simulink model "aero2_hardware_cascade_R2021a"  (R2021a)
settings: Solver=ode1  StartTime=0.0  StopTime=60  FixedStep=0.002  RelTol=1e-3  EnableMultiTasking=on
model workspace (MAT data in the model file):
  Dq = 2.25
  Kaw = 20
  Kff = 1
  Ki = 1.84164606325
  Kp = 0.216370391856
  Kq = 2.25
  ReferenceRate = [0 0.002 0.004 0.006 0.008 0.01 0.012 0.014 0.016 0.018 0.02 0.022 ... (90003 elements, 30001x3)]
  Ts = 0.002
  U_h : timeseries (value not decoded)
  U_v : timeseries (value not decoded)
  X0 = [0; 0; 0; 0]
  meas_on = 0
undefined symbols (not defined in the file): DiscIntNeverNeededParam, HIL, qc_get_step_size
libraries: quarc_library x4
(part 2 of 2)

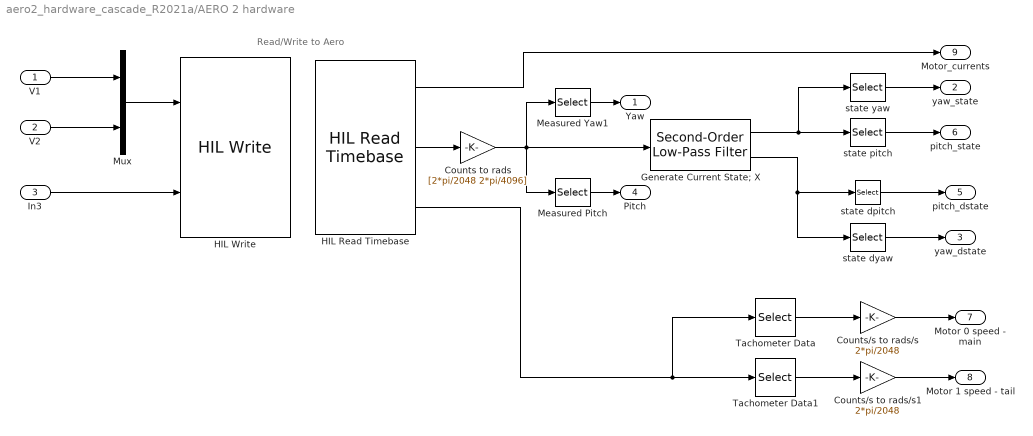
== system aero2_hardware_cascade_R2021a/AERO 2 hardware ==
  note: Read/Write to Aero
  V1 : Inport
  V2 : Inport  Port=2
  In3 : Inport  Port=3
  Counts to rads : Gain  Gain=[2*pi/2048 2*pi/4096]
  Counts/s to rads/s : Gain  Gain=2*pi/2048
  Counts/s to rads/s1 : Gain  Gain=2*pi/2048
  Generate Current State; X : quarc_library/Continuous/Second-Order Low-Pass Filter  params_source=Internal (dialog parameters)  input_width=10  input_zeta=0.8  input_init=0
  HIL Read Timebase : quarc_library/Data Acquisition/Generic/Timebases/HIL Read Timebase  object_name=HIL-1  clock=0  analog_channels=[0:1]  encoder_channels=[2:3]  digital_channels=[]  other_channels=[4000 4002 14000 14001]  active=on  vector_output=on  data_type_mode=Inherit via back propagation  encoder_data_type=double  digital_data_type=boolean  overflow_mode=Error on overflow  samples_in_buffer=max(ceil(1/qc_get_step_size), 1)
  HIL Write : quarc_library/Data Acquisition/Generic/Immediate I//O/HIL Write  object_name=HIL-1  analog_channels=[0:1]  pwm_channels=[]  digital_channels=[]  other_channels=[11000:11002]  sample_time=-1  active=off  vector_input=on
  Measured Pitch : Selector  InputPortWidth=2  IndexOptions=Index vector (dialog)  Indices=[1]  OutputSizes=1
  Measured Yaw1 : Selector  InputPortWidth=2  IndexOptions=Index vector (dialog)  Indices=[2]  OutputSizes=1
  Mux : Mux  Inputs=2
  Tachometer Data : Selector  InputPortWidth=4  IndexOptions=Index vector (dialog)  Indices=[3]  OutputSizes=1
  Tachometer Data1 : Selector  InputPortWidth=4  IndexOptions=Index vector (dialog)  Indices=[4]  OutputSizes=1
  state dpitch : Selector  InputPortWidth=2  IndexOptions=Index vector (dialog)  Indices=[1]  OutputSizes=1
  state dyaw : Selector  InputPortWidth=2  IndexOptions=Index vector (dialog)  Indices=[2]  OutputSizes=1
  state pitch : Selector  InputPortWidth=2  IndexOptions=Index vector (dialog)  Indices=[1]  OutputSizes=1
  state yaw : Selector  InputPortWidth=2  IndexOptions=Index vector (dialog)  Indices=[2]  OutputSizes=1
  Yaw : Outport
  yaw_state : Outport  Port=2
  yaw_dstate : Outport  Port=3
  Pitch : Outport  Port=4
  pitch_dstate : Outport  Port=5
  pitch_state : Outport  Port=6
  Motor 0 speed - main : Outport  Port=7
  Motor 1 speed - tail : Outport  Port=8
  Motor_currents : Outport  Port=9
  wires:
  Tachometer Data/1 -> Counts/s to rads/s/1
  HIL Read Timebase/3 -> Tachometer Data1/1, Tachometer Data/1
  Counts/s to rads/s1/1 -> Motor 1 speed - tail/1
  Tachometer Data1/1 -> Counts/s to rads/s1/1
  Counts/s to rads/s/1 -> Motor 0 speed - main/1
  Measured Yaw1/1 -> Yaw/1
  state dyaw/1 -> yaw_dstate/1
  state pitch/1 -> pitch_state/1
  Measured Pitch/1 -> Pitch/1
  V2/1 -> Mux/2
  state yaw/1 -> yaw_state/1
  HIL Read Timebase/1 -> Motor_currents/1
  Generate Current State; X/2 -> state dpitch/1, state dyaw/1
  In3/1 -> HIL Write/2
  HIL Read Timebase/2 -> Counts to rads/1
  Mux/1 -> HIL Write/1
  Counts to rads/1 -> Measured Yaw1/1, Generate Current State; X/1, Measured Pitch/1
  V1/1 -> Mux/1
  Generate Current State; X/1 -> state pitch/1, state yaw/1
  state dpitch/1 -> pitch_dstate/1

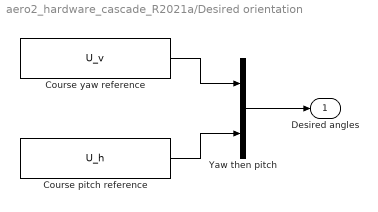
== system aero2_hardware_cascade_R2021a/Desired orientation ==
  Course pitch reference : FromWorkspace  VariableName=U_h  OutputAfterFinalValue=Holding final value
  Course yaw reference : FromWorkspace  VariableName=U_v  OutputAfterFinalValue=Holding final value
  Yaw then pitch : Mux  Inputs=2
  Desired angles : Outport
  wires:
  Course yaw reference/1 -> Yaw then pitch/1
  Course pitch reference/1 -> Yaw then pitch/2
  Yaw then pitch/1 -> Desired angles/1

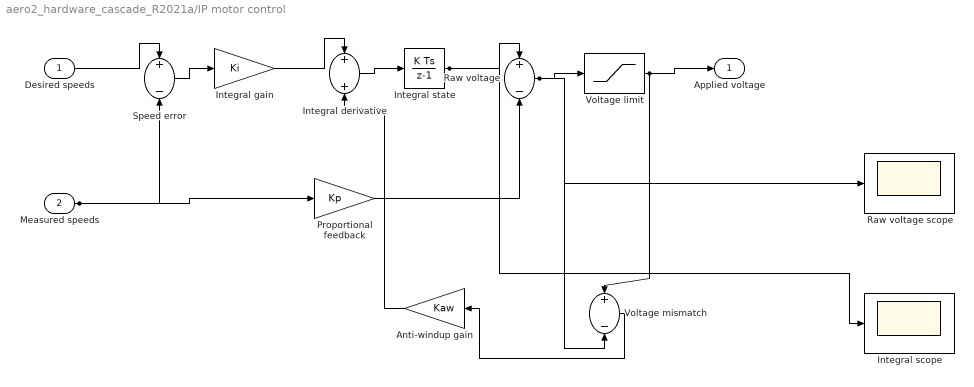
== system aero2_hardware_cascade_R2021a/IP motor control ==
  Desired speeds : Inport
  Measured speeds : Inport  Port=2
  Anti-windup gain : Gain  Gain=Kaw
  Integral derivative : Sum
  Integral gain : Gain  Gain=Ki
  Integral scope : Scope
  Integral state : DiscreteIntegrator  InitialCondition=[0;0]  SampleTime=Ts  ICPrevOutput=DiscIntNeverNeededParam  ICPrevScaledInput=DiscIntNeverNeededParam
  Proportional feedback : Gain  Gain=Kp
  Raw voltage : Sum  Inputs=+-
  Raw voltage scope : Scope
  Speed error : Sum  Inputs=+-
  Voltage limit : Saturate  UpperLimit=24  LowerLimit=-24
  Voltage mismatch : Sum  Inputs=+-
  Applied voltage : Outport
  wires:
  Desired speeds/1 -> Speed error/1
  Measured speeds/1 -> Speed error/2, Proportional feedback/1
  Speed error/1 -> Integral gain/1
  Integral gain/1 -> Integral derivative/1
  Proportional feedback/1 -> Raw voltage/2
  Raw voltage/1 -> Voltage limit/1, Voltage mismatch/2, Raw voltage scope/1
  Voltage limit/1 -> Applied voltage/1, Voltage mismatch/1
  Voltage mismatch/1 -> Anti-windup gain/1
  Anti-windup gain/1 -> Integral derivative/2
  Integral derivative/1 -> Integral state/1
  Integral state/1 -> Raw voltage/1, Integral scope/1

== matlab function aero2_hardware_cascade_R2021a/Mechanical inverse ==
  data: q input; omegaDesired output; dq input; a input
function omegaDesired = aero2_feedback_linearization(q, dq, a)
%AERO2_FEEDBACK_LINEARIZATION Ideal motor tracking: choose omega for q_ddot=a.
% The signed square root is defined at zero but has no finite derivative there.
p = aero2_mechanical_parameters;
assert(abs(q(2)) <= p.pitchLimit, 'Pitch envelope exceeded (limit 60 deg).');
[M, c, g, Gamma] = aero2_mechanical_terms(q, dq);
s = Gamma\(M*a+c+g);
omegaDesired = sign(s).*sqrt(abs(s));
end

function [M, c, g, Gamma] = aero2_mechanical_terms(q, dq)
%AERO2_MECHANICAL_TERMS M*q_ddot+c+g=Gamma*(omega.*abs(omega)).
% Signal order: q=[yaw;pitch], dq=[yaw rate;pitch rate], omega=[main;tail].
p = aero2_mechanical_parameters;
theta = q(2);
cor = p.Jyaw-p.jyaw;
M = [p.Jyaw*cos(theta)^2+p.jyaw*sin(theta)^2, 0; 0, p.Jpitch];
c = [-cor*sin(2*theta)*dq(2)*dq(1); ...
    0.5*cor*sin(2*theta)*dq(1)^2];
g = [0; p.gravity*sin(theta)];
Gamma = [cos(theta), 0; 0, 1]*[-p.kt, p.lever*p.kf; p.lever*p.kf, p.kt];
end

function p = aero2_mechanical_parameters
%AERO2_MECHANICAL_PARAMETERS Simplified course model, Part II, pages 4-5.
p.Jyaw = 0.6407;
p.jyaw = 0.01;
p.Jpitch = 0.7164;
p.gravity = 0.0254;
p.kt = 4.2487e-6;
p.kf = 2.5526e-5;
p.lever = 0.167;
p.pitchLimit = pi/3; % Simulation envelope, not an approved hardware limit.
p.initialState = [0.1; 0.2; -0.05; 0.04]; % [yaw; pitch; yaw rate; pitch rate].
p.acceleration = [0.15; -0.1];
p.step = 0.002;
end
